simulink model "FAFA_Simulation"  (R2024b)
settings: Solver=FixedStepAuto  StartTime=0.0  StopTime=250  FixedStep=0.1  RelTol=1e-3
model workspace (MAT data in the model file):
  E = 0
  N = 0
  U = 70
  a_lat = [-2.8994 -3.7694 4.8979 0.9075 0.2017 1.1605 -2.4536 1.8506 -1.4522 0.9879 -4.2099 6.4665 ... (16 elements, 4x4)]
  a_lon = [-0.1636 0.8185 -0.1448 0.6823 -0.7164 -0.2899 -2.0395 -2.5415 0.3908 2.1971 -0.2446 -6.117 ... (16 elements, 4x4)]
  b_lat = [-2.6641  1.8404; -6.8743  1.3852; 17.3529  -0.0089; -11.8089  -3.3692]
  b_lon = [1.3105; 2.2437; -0.9608; -9.211]
  c_lat = [-0.6923 -1.1619 0.5476 -0.4273 0.0805 0.5751 0.4203 0.7792 -0.3221 1.1098 0.2079 0.2479 ... (16 elements, 4x4)]
  c_lon = [-5.1576 -0.0952 0.5331 3.6707 -28.9963 -0.3715 -3.4973 -0.1414 19.7487 -0.0997 -0.5832 -0.2256 ... (16 elements, 4x4)]
  d_lat = [0  0; 0  0; 0  0; 0  0]
  d_lon = [0; 0; 0; 0]
  psi0 = 0
  wind_E0 = 0
  wind_N0 = 0
  wind_heading = 100
  wind_noise = 0
  wind_turbulance_value0 = 1
  wind_value0 = 0
  x0_lat = [0; 0; 0; 0]
  x0_lon = [0; 0; 0; 0]
values from neighbouring files (symbols this model uses):
  velocity = zeros(num_waypoints, 3)    [training_engine.m]
  waypoints = all_waypoints    [training_engine.m]
undefined symbols (not defined in the file or in its folder): dspblkCoreblockFVToolHelper, F, gcbh, Light, MIL
libraries: simulink x8, slpidlib x5, aerolibwind2 x3, sharedtransform x2, rllib x1, uavutilslib x1
(part 2 of 3)

== matlab function FAFA_Simulation/OBSERVATION/MATLAB Function8 ==
  data: waypoints_window input; velocity_window input; valid_flag input; loiter_flag input; uav_e input; global_path output size=[inf 3]; uav_n input; uav_u input; guidance_mode output; uav_phi input; uav_theta input; uav_psi input
function [global_path, guidance_mode]   = guidance_function_hybrid(waypoints_window, velocity_window, valid_flag, loiter_flag, uav_e, uav_n, uav_u, uav_phi, uav_theta, uav_psi)

% guidance_mode: 0=無效, 1=純B-spline, 2=SPSO+B-spline, 3=Loiter模式

%#codegen

%  Loiter 模式開關
ENABLE_LOITER = false;

persistent last_point_initialized last_point stored_global_path stored_path_length ...
           loiter_mode initialized theta_current center loiter_arc transition

if isempty(last_point_initialized)
    last_point_initialized = false;
    last_point            = zeros(1,3);
    stored_global_path    = zeros(100000,3);
    stored_path_length    = 1;
    loiter_mode           = false;
    initialized = false;
    theta_current = 0;
    center = [0 0];
    loiter_arc = zeros(3,3);  % 固定初始大小
    transition = false;
end

% 確保 guidance_mode 在所有路徑都有明確的標量值
guidance_mode = 0;

R = 100;
dtheta_deg = 1;
uav_position = [uav_e, uav_n, uav_u];

%% ==== Loiter 模式 ====
% 只有當 ENABLE_LOITER = true 時才會進入 Loiter 邏輯
if ENABLE_LOITER && loiter_flag && ~initialized
    if stored_path_length >= 2
        pos_prev = stored_global_path(stored_path_length-1, 1:2);
        pos_curr = stored_global_path(stored_path_length, 1:2);
        heading_vec = pos_curr - pos_prev;
        yaw = atan2(heading_vec(2), heading_vec(1));
    else
        yaw = 0;
    end
    
    dists = vecnorm(waypoints_window(:,1:2) - uav_position(1:2), 2, 2);
    [~, idx_nearest] = min(dists);
    P0 = waypoints_window(idx_nearest, 1:2);
    center = P0 + [cos(yaw), sin(yaw)] * R * 1.5;
    theta_current = atan2(uav_position(2) - center(2), ...
                           uav_position(1) - center(1));
    loiter_mode = true;
    initialized = true;
end

if ENABLE_LOITER && loiter_mode
    guidance_mode = 3;
    if loiter_flag
        dtheta = deg2rad(dtheta_deg);
        spacing = 1.0;
        arc_length = R * dtheta;
        num_points = max(3, ceil(arc_length / spacing));
        theta_list = theta_current - linspace(0, dtheta, num_points);
        x_list = center(1) + R * cos(theta_list);
        y_list = center(2) + R * sin(theta_list);
        z_list = repmat(uav_u, size(x_list));

        loiter_arc_raw = [x_list', y_list', z_list'];
        arc_diff = diff(loiter_arc_raw);
        arc_seg_length = sqrt(sum(arc_diff.^2, 2));
        cum_length = [0; cumsum(arc_seg_length)];
        total_length = cum_length(end);

        num_interp = max(2, ceil(total_length));
        query_dist = linspace(0, total_length, num_interp)';
        interp_x = interp1(cum_length, loiter_arc_raw(:,1), query_dist, 'linear');
        interp_y = interp1(cum_length, loiter_arc_raw(:,2), query_dist, 'linear');
        interp_z = interp1(cum_length, loiter_arc_raw(:,3), query_dist, 'linear');
        loiter_arc = [interp_x, interp_y, interp_z];
        theta_current = theta_list(end);

        if ~transition
            loiter_entry = loiter_arc(1,:);
            loiter_tangent = loiter_arc(2,1:2) - loiter_arc(1,1:2);
            loiter_tangent = loiter_tangent / (norm(loiter_tangent) + 1e-6);

            dists = vecnorm(waypoints_window(:,1:2) - uav_position(1:2), 2, 2);
            [~, idx_nearest] = min(dists);
            P0 = waypoints_window(idx_nearest, :);
            
            connect_tangent = loiter_entry(1:2) - P0(1:2);
            connect_tangent = connect_tangent / (norm(connect_tangent) + 1e-6);
            dist = norm(loiter_entry(1:2) - P0(1:2));

            P1 = P0(1:2) + 0.3 * dist * connect_tangent;
            P2 = loiter_entry(1:2) - 0.3 * dist * loiter_tangent;
            P3 = loiter_entry(1:2);

            t = linspace(0,1,ceil(dist));
            bezier_x = (1-t).^3 * P0(1) + 3*(1-t).^2 .* t * P1(1) + 3*(1-t).*t.^2 * P2(1) + t.^3 * P3(1);
            bezier_y = (1-t).^3 * P0(2) + 3*(1-t).^2 .* t * P1(2) + 3*(1-t).*t.^2 * P2(2) + t.^3 * P3(2);
            bezier_z = linspace(P0(3), loiter_entry(3), numel(t));
            transition_path = [bezier_x', bezier_y', bezier_z'];

            combined_path = [transition_path; loiter_arc(2:end,:)];
            global_path = combined_path;
            transition = true;
        else
            global_path = loiter_arc;
        end
        return;
    else
        % 退出 Loiter 的邏輯
        arc_exit_pt = loiter_arc(end, :);
        arc_tangent = loiter_arc(end,1:2) - loiter_arc(end-1,1:2);
        arc_tangent = arc_tangent / (norm(arc_tangent) + 1e-6);
        R_min = 55;
        dists = vecnorm(waypoints_window(:,1:2) - arc_exit_pt(1:2), 2, 2);
        [~, idx_nearest] = min(dists);
        lookahead_distance = 100;
        accum_dist = 0;
        idx_target = idx_nearest;
        while accum_dist < lookahead_distance && idx_target < size(waypoints_window,1)
            delta = norm(waypoints_window(idx_target+1,1:2) - waypoints_window(idx_target,1:2));
            accum_dist = accum_dist + delta;
            idx_target = idx_target + 1;
        end
        p_target = waypoints_window(idx_target, :);
        if idx_target < size(waypoints_window,1)
            next_vec = waypoints_window(idx_target+1,1:2) - waypoints_window(idx_target,1:2);
        else
            next_vec = waypoints_window(idx_target,1:2) - waypoints_window(idx_target-1,1:2);
        end
        target_tangent = next_vec / (norm(next_vec) + 1e-6);
        P0 = arc_exit_pt;
        P3 = p_target;
        total_dist = norm(P3(1:2) - P0(1:2));
        theta = acos(dot(arc_tangent, target_tangent));
        d_min = R_min * tan(theta/2);
        d = max(d_min, R_min);
        success = false;
        B = repmat(P0, ceil(total_dist), 1);
        while ~success && d <= total_dist
            P1 = P0 + [arc_tangent, 0] * 0.3 * d;
            P2 = P3 - [target_tangent, 0] * 0.1 * d;
            t = linspace(0,1,ceil(total_dist));
            B = (1 - t').^3 * P0 + 3*(1 - t').^2 .* t' * P1 + 3*(1 - t') .* t'.^2 * P2 + t'.^3 * P3;
            d1 = diff(B, 1, 1);
            d2 = diff(d1, 1, 1);
            cross_z = d1(1:end-1,1) .* d2(:,2) - d1(1:end-1,2) .* d2(:,1);
            curvature = abs(cross_z) ./ (vecnorm(d1(1:end-1,:),2,2).^3 + 1e-6);
            if all(1./(curvature + 1e-6) >= R_min)
                success = true;
            else
                d = d + 5;
            end
        end
        segment = B;
        stored_global_path(1:size(segment,1), :) = segment;
        stored_path_length = size(segment,1);
        loiter_mode = false;
        initialized = false;
        transition = false;
        global_path = segment;
        % 固定維度賦值
        if size(segment,1) >= 1
            last_point(1,1) = segment(end, 1);
            last_point(1,2) = segment(end, 2);
            last_point(1,3) = segment(end, 3);
        end
        return;
    end
end

%% ========== v8 混合規劃器 ==========
if valid_flag && ~loiter_mode
    
    N_WAYPOINTS = size(waypoints_window, 1);
    
    % 起點處理 
    if ~last_point_initialized
        P_start_spline = [uav_e, uav_n, uav_u];
        last_point_initialized = true;
    else
        P_start_spline = last_point;
    end
    
    P_end = waypoints_window(end, :);

    % 判斷模式
    % dists_to_window = vecnorm(waypoints_window - uav_position, 2, 2);             % 三維距離
    dists_to_window = vecnorm(waypoints_window(:,1:2) - uav_position(1:2), 2, 2);   % 水平距離

    [min_dist_to_window, ~] = min(dists_to_window);
    % dist_start_to_window = norm(P_start_spline - waypoints_window(1,:));          % 三維距離
    dist_start_to_window = norm(P_start_spline(1:2) - waypoints_window(1,1:2));     % 水平距離

    DEVIATION_THRESHOLD = 100;  
    
    if min_dist_to_window < DEVIATION_THRESHOLD && dist_start_to_window < DEVIATION_THRESHOLD
        % ========== 模式A：純B-spline  ==========
        guidance_mode = 1;
        N_CONTROL_POINTS = 6;
        indices = round(linspace(1, N_WAYPOINTS, N_CONTROL_POINTS));
        best_control_points = waypoints_window(indices, :);
        best_control_points(1, :) = P_start_spline; 
    else
        % ========== 模式B：SPSO + B-spline ==========
        guidance_mode = 2;
        
        % SPSO 起點：強制為 UAV 當前位置
        P_start_SPSO = uav_position;
        
        % ====== 目標行駛方向（由速度滑窗估計，僅 SPSO 使用） ======
        v_tar_2d = [0, 0];
        if ~isempty(velocity_window)
            N_vel = size(velocity_window, 1);
            if N_vel >= 1
                K = min(3, N_vel);                    % 用最後 3 筆速度平均
                idx_start = N_vel - K + 1;
                v_seg = velocity_window(idx_start:N_vel, 1:2); % 只取 [vx, vy]
                v_mean = mean(v_seg, 1);
                if norm(v_mean) > 1e-3
                    v_tar_2d = v_mean;
                else
                    v_tar_2d = [0, 0];                % 速度太小則視為無效，不啟用角度限制
                end
            end
        end
        
        % SPSO參數
        nParticles = 10;
        maxIter = 20;
        w = 0.4;
        c1 = 1.5;
        c2 = 1.5;
        
        N_CONTROL_POINTS = 5; % 起點(UAV) + 3中間 + 終點
        N_OPTIMIZE = 3;
        
        % 定義 SPSO 粒子空間限制 (無人機運動學限制)
        % 直接限制粒子生成範圍
        max_segment_length = 50;
        min_segment_length = 5;
        max_climb_angle_rad = deg2rad(20); % 限制爬升角 theta
        % SPSO 粒子方位角相對轉角限制
        max_turn_angle_rad  = deg2rad(35); 
        
        % 權重設定 (總和 = 1)
        % b1: 路徑長度 (Shortest Path)
        % b2: 路徑跟隨 (Tracking)
        % b3: 平滑度 (Smoothness)
        % b4: 終點誤差 (Endpoint)
        b1 = 0.6; 
        b2 = 0.2; 
        b3 = 0.1; 
        b4 = 0.1; 

        % 參考採樣
        sample_idx = round(linspace(1, N_WAYPOINTS, N_CONTROL_POINTS));
        control_waypoints = waypoints_window(sample_idx, :);
        
        % 初始化參考向量 (基於 UAV 位置)
        reference_vectors = control_waypoints - P_start_SPSO;
        rho_ref = vecnorm(reference_vectors, 2, 2);
        theta_ref = asin(reference_vectors(:,3) ./ (rho_ref + 1e-6));
        phi_ref = atan2(reference_vectors(:,2), reference_vectors(:,1));
        
        dim = N_OPTIMIZE * 3;
        particles = zeros(nParticles, dim);
        velocities = zeros(nParticles, dim);
        
        for i = 1:nParticles
            for j = 1:N_OPTIMIZE
                ref_idx = j + 1;
                idx = (j-1)*3 + 1;
                
                if i == 1
                    % 第一個粒子用參考值
                    particles(1, idx)   = rho_ref(ref_idx);
                    particles(1, idx+1) = theta_ref(ref_idx);
                    particles(1, idx+2) = phi_ref(ref_idx);
                else
                    % 隨機生成
                    particles(i, idx)   = rho_ref(ref_idx) * (1 + randn() * 0.1);
                    particles(i, idx+1) = theta_ref(ref_idx) + randn() * deg2rad(2);
                    particles(i, idx+2) = phi_ref(ref_idx) + randn() * deg2rad(5);
                end
                
                % 在生成階段強制限制範圍
                % 限制長度 rho
                particles(i, idx) = max(min_segment_length, min(particles(i, idx), max_segment_length));
                % 限制爬升角 theta (直接對應無人機 Pitch/Climb 限制)
                particles(i, idx+1) = max(-max_climb_angle_rad, min(particles(i, idx+1), max_climb_angle_rad));
                
                % 限制方位角 phi 的「相對轉角」在 ±max_turn_angle_rad 內
                if j == 1
                    % 第一段以 UAV 目前航向為基準
                    base_heading = uav_psi;
                else
                    % 之後每一段以「前一段的 phi」為基準
                    prev_phi_idx = (j-2)*3 + 3;
                    base_heading = particles(i, prev_phi_idx);
                end
                dphi = particles(i, idx+2) - base_heading;
                % 將角度包回 [-pi, pi]
                dphi = mod(dphi + pi, 2*pi) - pi;
                % 夾住相對轉角
                if dphi > max_turn_angle_rad
                    dphi = max_turn_angle_rad;
                elseif dphi < -max_turn_angle_rad
                    dphi = -max_turn_angle_rad;
                end
                % 更新 phi 並保持在 [-pi, pi]
                particles(i, idx+2) = mod(base_heading + dphi + pi, 2*pi) - pi;
            end
            velocities(i, :) = randn(1, dim) * 0.01;
        end
        
        % SPSO迭代 - 初始 fitness
        fitness = zeros(nParticles, 1);
        for i = 1:nParticles
            % 傳入 uav_psi 以及 v_tar_2d 以計算初始航向與終端入射角
            fitness(i) = evaluateFitness_CostStruct(particles(i,:), P_start_SPSO, P_end, ...
                          control_waypoints, N_CONTROL_POINTS, b1, b2, b3, b4, ...
                          uav_psi, v_tar_2d);
        end
        
        [~, best_idx] = min(fitness);
        personal_best = particles;
        personal_best_fitness = fitness;
        global_best = particles(best_idx, :);
        global_best_fitness = fitness(best_idx);
        
        for iter = 1:maxIter
            for i = 1:nParticles
                r1 = rand(1, dim);
                r2 = rand(1, dim);
                velocities(i,:) = w * velocities(i,:) + ...
                                  c1 * r1 .* (personal_best(i,:) - particles(i,:)) + ...
                                  c2 * r2 .* (global_best - particles(i,:));
                particles(i,:) = particles(i,:) + velocities(i,:);
                
                % 更新後再次強制限制範圍 (Constraints)
                for j = 1:N_OPTIMIZE
                    idx = (j-1)*3 + 1;
                    % Rho Constraint
                    particles(i, idx) = max(min_segment_length, min(particles(i, idx), max_segment_length));
                    % Theta Constraint (Climb Angle)
                    particles(i, idx+1) = max(-max_climb_angle_rad, min(particles(i, idx+1), max_climb_angle_rad));
                    
                    % Phi Constraint: 限制每段方位角相對前一段 / UAV 航向的轉角
                    phi_idx = idx + 2;
                    if j == 1
                        base_heading = uav_psi;
                    else
                        prev_phi_idx = (j-2)*3 + 3;
                        base_heading = particles(i, prev_phi_idx);
                    end
                    dphi = particles(i, phi_idx) - base_heading;
                    % 將角度包回 [-pi, pi]
                    dphi = mod(dphi + pi, 2*pi) - pi;
                    % 夾住相對轉角
                    if dphi > max_turn_angle_rad
                        dphi = max_turn_angle_rad;
                    elseif dphi < -max_turn_angle_rad
                        dphi = -max_turn_angle_rad;
                    end
                    % 更新 phi 並保持在 [-pi, pi]
                    particles(i, phi_idx) = mod(base_heading + dphi + pi, 2*pi) - pi;
                end

                fitness(i) = evaluateFitness_CostStruct(particles(i,:), P_start_SPSO, P_end, ...
                              control_waypoints, N_CONTROL_POINTS, b1, b2, b3, b4, ...
                              uav_psi, v_tar_2d);

                if fitness(i) < personal_best_fitness(i)
                    personal_best(i,:) = particles(i,:);
                    personal_best_fitness(i) = fitness(i);
                end
            end
            
            [current_best_fitness, best_idx] = min(fitness);
            if current_best_fitness < global_best_fitness
                global_best = particles(best_idx, :);
                global_best_fitness = current_best_fitness;
            end
        end
        
        % 構建最終控制點
        best_control_points = zeros(N_CONTROL_POINTS, 3);
        best_control_points(1, :) = P_start_SPSO; 
        best_control_points(end, :) = P_end;
        for j = 1:N_OPTIMIZE
            idx = (j-1)*3 + 1;
            rho   = global_best(idx);
            theta = global_best(idx+1);
            phi   = global_best(idx+2);
            dx = rho * cos(theta) * cos(phi);
            dy = rho * cos(theta) * sin(phi);
            dz = rho * sin(theta);
            best_control_points(j+1, :) = best_control_points(j, :) + [dx, dy, dz];
        end
    end
    
    % 生成 B-spline
    N_samples = 100;
    path_smooth = generate_Bspline(best_control_points, N_samples);
    
    % Resample
    segment_diff = diff(path_smooth);
    segment_length = sqrt(sum(segment_diff.^2, 2));
    cumulative_length = [0; cumsum(segment_length)];
    total_length = cumulative_length(end);
    
    if total_length < 1e-3
        if stored_path_length > 1
             global_path = stored_global_path(1:stored_path_length,:);
        else
             global_path = path_smooth;
        end
        return;
    end
    
    desired_spacing = 1;
    num_new_points = max(2, floor(total_length / desired_spacing));
    query_distances = linspace(0, total_length, num_new_points)';
    
    interp_x = interp1(cumulative_length, path_smooth(:,1), query_distances, 'linear');
    interp_y = interp1(cumulative_length, path_smooth(:,2), query_distances, 'linear');
    interp_z = interp1(cumulative_length, path_smooth(:,3), query_distances, 'linear');
    
    new_path = [interp_x, interp_y, interp_z];
    stored_global_path(:,:) = 0;
    if isempty(new_path)
        stored_global_path(1:size(best_control_points,1),:) = best_control_points;
        stored_path_length = size(best_control_points,1);
        % 固定維度賦值
        last_point(1,1) = best_control_points(end, 1);
        last_point(1,2) = best_control_points(end, 2);
        last_point(1,3) = best_control_points(end, 3);
    else
        stored_global_path(1:size(new_path,1),:) = new_path;
        stored_path_length = size(new_path,1);
        % 固定維度賦值
        last_point(1,1) = new_path(end, 1);
        last_point(1,2) = new_path(end, 2);
        last_point(1,3) = new_path(end, 3);
    end
end

global_path = stored_global_path(1:stored_path_length,:);
end

%% ========== B-spline生成器 ==========
function path_smooth = generate_Bspline(control_points, num_samples)
    N = size(control_points, 1);
    if N < 2
        path_smooth = control_points;
        return;
    end
    segment_lengths = sqrt(sum(diff(control_points).^2, 2));
    t_control = [0; cumsum(segment_lengths)];
    valid_idx = [true; segment_lengths > 1e-6];
    if sum(valid_idx) < 2
        path_smooth = repmat(control_points(1,:), num_samples, 1);
        return;
    end
    t_control_valid = t_control(valid_idx);
    control_points_valid = control_points(valid_idx, :);
    if isempty(t_control_valid) || t_control_valid(end) < 1e-6
        path_smooth = repmat(control_points(1,:), num_samples, 1);
        return;
    end
    t_control_valid = t_control_valid / t_control_valid(end); 
    t_query = linspace(0, 1, num_samples)';
    x_smooth = spline(t_control_valid, control_points_valid(:,1), t_query);
    y_smooth = spline(t_control_valid, control_points_valid(:,2), t_query);
    z_smooth = spline(t_control_valid, control_points_valid(:,3), t_query);
    path_smooth = [x_smooth, y_smooth, z_smooth];
end

%% ========== Cost Function（含終端入射角約束） ==========
function cost = evaluateFitness_CostStruct(particle, P_start, P_end, control_waypoints, N_control, ...
                                           b1, b2, b3, b4, ...
                                           uav_psi, v_tar_2d)
    % particle: SPSO 粒子向量
    % b1: Shortest Path (長度)
    % b2: Tracking (跟隨誤差)
    % b3: Smoothness (平滑度 & 初始姿態限制)
    % b4: Endpoint (終點誤差)
    % v_tar_2d: 目標行駛方向（由速度滑窗估計）[vx, vy]
    
    % 1. 重建路徑 (SPSO 控制點)
    path = zeros(N_control, 3);
    path(1, :) = P_start;
    path(end, :) = P_end;
    
    N_optimize = (N_control - 2);
    for j = 1:N_optimize
        idx = (j-1)*3 + 1;
        rho   = particle(idx);
        theta = particle(idx+1);
        phi   = particle(idx+2);
        dx = rho * cos(theta) * cos(phi);
        dy = rho * cos(theta) * sin(phi);
        dz = rho * sin(theta);
        path(j+1, :) = path(j, :) + [dx, dy, dz];
    end
    
    % ========== F1: 路徑長度成本 (Shortest Path) ==========
    path_diff = diff(path);
    segment_lengths = sqrt(sum(path_diff.^2, 2));
    total_length = sum(segment_lengths);
    straight_dist = norm(P_end - P_start);
    
    if straight_dist > 1e-6
        F1 = total_length / straight_dist; % 越接近1越好
        F1 = min(F1, 3.0); % 上限截斷
    else
        F1 = 1.0;
    end
    
    % ========== F2: 路徑跟隨成本 (Tracking) ==========
    F2_raw = 0;
    for i = 1:size(path,1)
        dists = vecnorm(control_waypoints - path(i,:), 2, 2);
        [min_dist, ~] = min(dists);
        F2_raw = F2_raw + min_dist^2; % 平方懲罰
    end
    F2 = F2_raw / (size(path,1) * 100); % 簡單歸一化
    F2 = min(F2, 10.0);

    % ========== F3: 平滑度成本 (Smoothness & UAV Heading) ==========
    F3_raw = 0;
    max_turn_angle = deg2rad(35);
    
    % (A) 檢查第一段路徑與 UAV 當前航向 (psi) 的夾角
    vec_first = path(2,1:2) - path(1,1:2);
    if norm(vec_first) > 1e-6
        current_psi_vec = [cos(uav_psi), sin(uav_psi)];
        dot_val = dot(vec_first/norm(vec_first), current_psi_vec);
        angle_diff_start = acos(max(-1, min(1, dot_val)));
        
        % 如果起步轉彎大於限制，給予巨大懲罰
        if angle_diff_start > max_turn_angle
            cost = 1e9; 
            return;
        end
        F3_raw = F3_raw + angle_diff_start;
    end
    
    % (B) 檢查後續路徑段之間的夾角
    for i = 1:size(path,1)-2
        v1 = path(i+1,1:2) - path(i,1:2);
        v2 = path(i+2,1:2) - path(i+1,1:2);
        
        if norm(v1) > 1e-6 && norm(v2) > 1e-6
            dot_prod = dot(v1, v2);
            cross_prod = v1(1)*v2(2) - v1(2)*v2(1);
            phi_turn = atan2(cross_prod, dot_prod);
            
            if abs(phi_turn) > max_turn_angle
                cost = 1e9;
                return;
            end
            F3_raw = F3_raw + abs(phi_turn);
        end
    end
    F3 = F3_raw; % 可根據需要添加歸一化因子
    
    % ========== F4: 終點誤差成本 (Endpoint) ==========
    endpoint_error = norm(path(end,:) - P_end);
    if endpoint_error > 20 % 硬約束寬鬆一點給 SPSO
        cost = 1e9 + endpoint_error * 1000;
        return;
    end
    F4 = endpoint_error / 10.0;
    
    % ========== F5: 終端入射角成本（硬約束：±45°） ==========
    % 僅當 v_tar_2d 有效時啟用（速度非接近 0）
    if ~(v_tar_2d(1) == 0 && v_tar_2d(2) == 0)
        if size(path,1) < 2
            cost = 1e9;
            return;
        end
        
        % 終端路徑的切線向量（水平平面）
        v_last = path(end,1:2) - path(end-1,1:2);
        if norm(v_last) < 1e-6
            cost = 1e9;
            return;
        end
        v_last = v_last / norm(v_last);
        
        % 目標行駛方向向量正規化
        v_tar = v_tar_2d;
        if norm(v_tar) < 1e-6
            % 如果這裡還是太小，就不啟用此約束
        else
            v_tar = v_tar / norm(v_tar);
            
            % 入射角：終端切線 vs 目標行駛方向
            dot_val   = dot(v_last, v_tar);
            dot_val   = max(-1, min(1, dot_val));
            cross_val = v_last(1)*v_tar(2) - v_last(2)*v_tar(1);
            delta_psi_entry = atan2(cross_val, dot_val);  % [-pi, pi]
            
            max_entry = deg2rad(45); % 入射角限制 ±45°
            if abs(delta_psi_entry) > max_entry
                cost = 1e9;
                return;
            end
        end
    end

    % ========== 總成本 ==========
    cost = b1*F1 + b2*F2 + b3*F3 + b4*F4;
    
    if isnan(cost) || isinf(cost)
        cost = 1e10;
    end
end

== matlab function FAFA_Simulation/OBSERVATION/MATLAB Function10 ==
  data: x input; y output; finite input
function y = Normalization(x,finite)
y = (x-(-finite))/(finite-(-finite))*2-1;

== matlab function FAFA_Simulation/OBSERVATION/MATLAB Function9 ==
  data: x input; y output; finite input
function y = Normalization(x,finite)
y = (x-(-finite))/(finite-(-finite))*2-1;

== matlab function FAFA_Simulation/OBSERVATION/MATLAB Function13 ==
  data: kt input; y output; d input
function y = fcn(kt, d)

if abs(kt) >= (1/55)
    y = 0.5 *d;
else
    y = d;
end

== matlab function FAFA_Simulation/OBSERVATION/MATLAB Function11 ==
  data: x input; y output; finite input
function y = Normalization(x,finite)
y = (x-(-finite))/(finite-(-finite))*2-1;

== matlab function FAFA_Simulation/OBSERVATION/MATLAB Function12 ==
  data: E output; P_N input; N output; P_E input; psi input; v input; path input; d output; delta_psi output; heta output; curvature output; windowLen input
function [E, N, d, delta_psi, heta, curvature] = guidance_law(P_N, P_E, psi, v, path, windowLen)

    persistent global_path path_length last_path old_length heta_filt
    
    if isempty(global_path)
        global_path = zeros(500000, 3);
        path_length = 0;
        last_path = zeros(500000, 3);
        old_length = 0;
        heta_filt = 0;
    end
    
    % 如果這次輸入的 path 不等於上次的，就加入累積
    if ~isempty(path) && ~isequal(path, last_path(1:old_length, :))
        new_len = size(path, 1);
        global_path(path_length+1:path_length+new_len, :) = path(:, :);
        path_length = path_length + new_len;
        last_path(1:new_len, :) = path(:, :);
        old_length = new_len;
    end
    path_CTE = global_path(1:path_length, :);

    r = 0;
    curvature = 0;
    d = 0;
    delta_psi = 0;
    heta = 0;

    % Use the waypoints in the given path
    numWps = size(path, 1);
    if numWps < 2
        N = P_N;
        E = P_E;
        return;
    end

    % ============================================================
    % 前瞻曲率（用滑窗 path 末端那一段來估）
    % ============================================================
    if numWps < 3
        curvature = 0;
    else
        % 調這兩個 
        previewDist = 0.9 * windowLen;  % 看視野最前端附近（90%處） 300*0.9=270
        spanDist    = max(10, 0.1 * windowLen); % 用 10%視野估曲率，至少10m,270*0.1=27,計算270m前後27m的曲率
        % ------------------------

        % 以 path 起點為 0，計算沿路徑累積距離（平面 E,N）
        xy = path(:,1:2);
        s  = [0; cumsum(sqrt(sum(diff(xy).^2,2)))];  % s(i) = 第 i 點距離 path(1) 的弧長
        L  = s(end);

        if L < 1e-6
            curvature = 0;
        else
            % 把 previewDist 限制在滑窗長度內
            s2 = min(max(previewDist, 0), L);
            s1 = max(s2 - spanDist/2, 0);
            s3 = min(s2 + spanDist/2, L);

            % 找到最接近 s1,s2,s3 的三個點索引
            [~, i1] = min(abs(s - s1));
            [~, i2] = min(abs(s - s2));
            [~, i3] = min(abs(s - s3));

            % 確保三點不重疊（避免除0）
            if numel(unique([i1 i2 i3])) < 3
                curvature = 0;
            else
                A = xy(i1,:); B = xy(i2,:); C = xy(i3,:);

                a = norm(B - C);
                b = norm(A - C);
                c = norm(A - B);

                % signed area2 = 2*Area (帶正負號可分左右轉)
                area2 = (B(1)-A(1))*(C(2)-A(2)) - (B(2)-A(2))*(C(1)-A(1));

                if a*b*c < 1e-9 || abs(area2) < 1e-9
                    curvature = 0;
                    r = 0;
                else
                    curvature = (2 * area2) / (a*b*c);   % signed curvature (1/m)
                    r = 1 / max(abs(curvature), 1e-9);
                end
            end
        end
    end
    % ============================================================

    margin = 30;  
    min_E = min(path(:,1)) - margin;
    max_E = max(path(:,1)) + margin;
    min_N = min(path(:,2)) - margin;
    max_N = max(path(:,2)) + margin;

    is_inside = (P_E >= min_E) && (P_E <= max_E) && ...
            (P_N >= min_N) && (P_N <= max_N);

    if is_inside
        extended_P = repmat([P_E, P_N], numWps, 1);
        differences = path(:, 1:2) - extended_P;
        distances = sqrt(sum(differences.^2, 2));
        
        % Find the closest waypoint
        [~, current_index] = min(distances);
        
        % Define target distance
        target_distance = 50;
        
        % Compute cumulative distances
        cumulative_distances = [0; cumsum(sqrt(sum(diff(path).^2, 2)))];
        remaining_distances = cumulative_distances(current_index+1:end) - cumulative_distances(current_index);
        
        % Determine target index
        if isempty(remaining_distances) || current_index + 1 > numWps
            k = numWps;
        else
            % Find the waypoint at the target distance
            [~, target_index_offset] = min(abs(remaining_distances - target_distance));
            
            if current_index + target_index_offset > numWps
                k = numWps;
            else
                k = current_index + target_index_offset;
            end
        end
        
        % Target waypoint
        N = path(k, 2); 
        E = path(k, 1); 
    
        % Compute cross-track error
        if current_index >= numWps
            x1 = path(numWps-1, 1);
            y1 = path(numWps-1, 2);
            x2 = path(numWps, 1);
            y2 = path(numWps, 2);
        else
            x1 = path(current_index, 1);
            y1 = path(current_index, 2);
            x2 = path(current_index+1, 1);
            y2 = path(current_index+1, 2);
        end
        
        D = sqrt((P_N - y1)^2 + (P_E - x1)^2);
        psi_r = atan2(y2 - y1, x2 - x1);
        psi_c = atan2(P_N - y1, P_E - x1);
    
        if abs(psi_r - psi_c) < 1e-3
            d = 0; % 避免極小角度導致大誤差
        else
            d = abs(D * sin(psi_r - psi_c));
        end
           
        % Evaluation candidate: extend terminal lookahead while waiting for a new path.
        % Only the inside-window branch and its endpoint target are affected.
        if k == numWps
            tail = path(numWps,1:2) - path(numWps-1,1:2);
            tail_length = norm(tail);
            if tail_length > 1e-6
                tangent = tail / tail_length;
                along = dot([P_E, P_N] - path(numWps,1:2), tangent);
                extension = max(0, target_distance + along);
                E = path(numWps,1) + extension*tangent(1);
                N = path(numWps,2) + extension*tangent(2);
            end
        end

        % Compute heading difference
        psi_cmd = atan2(N - P_N, E - P_E);
        heta = psi_cmd - psi;
        heta = mod(heta + pi, 2 * pi) - pi;
    
        L1 = sqrt((N - P_N)^2 + (E - P_E)^2);
        a_cmd = 2 * v^2 / L1 * sin(heta);
        delta_psi = a_cmd / v;

    else  % ~is_inside
        
        numWaypoints = size(path_CTE, 1);
        % Calculate distances to all waypoints
        extended_P = repmat([P_E, P_N], numWaypoints, 1);
        differences = path_CTE(:, 1:2) - extended_P;
        distances = sqrt(sum(differences.^2, 2));
        
        % Find the closest waypoint
        [~, current_index] = min(distances);
        
        % Define target distance
        target_distance = 30;
        uav_pos = [P_E, P_N];
        path_points = path(:,1:2);
        point_dists = vecnorm(path_points - uav_pos, 2, 2);
        [~, k] = min(abs(point_dists - target_distance));
        
        % Target waypoint
        E = path(k, 1); 
        N = path(k, 2); 
    
        % Compute cross-track error
        if current_index >= numWaypoints
            x1 = path_CTE(numWaypoints-1, 1);
            y1 = path_CTE(numWaypoints-1, 2);
            x2 = path_CTE(numWaypoints, 1);
            y2 = path_CTE(numWaypoints, 2);
        else
            x1 = path_CTE(current_index, 1);
            y1 = path_CTE(current_index, 2);
            x2 = path_CTE(current_index+1, 1);
            y2 = path_CTE(current_index+1, 2);
        end
        
        D = sqrt((P_N - y1)^2 + (P_E - x1)^2);
        psi_r = atan2(y2 - y1, x2 - x1);
        psi_c = atan2(P_N - y1, P_E - x1);
    
        if abs(psi_r - psi_c) < 1e-3
            d = 0; % 避免極小角度導致大誤差
        else
            d = abs(D * sin(psi_r - psi_c));
        end
    
        % V2: only handle longitudinal overshoot near the terminal ray.
        tail = path(numWps,1:2) - path(numWps-1,1:2);
        tail_length = norm(tail);
        if tail_length > 1e-6
            tangent = tail / tail_length;
            offset = [P_E, P_N] - path(numWps,1:2);
            along = dot(offset, tangent);
            lateral = norm(offset - along*tangent);
            [~, nearest_terminal] = min(point_dists);
            if nearest_terminal == numWps && along >= 0 && lateral <= margin
                E = path(numWps,1) + (along + 50)*tangent(1);
                N = path(numWps,2) + (along + 50)*tangent(2);
            end
        end

        % Compute heading difference
        psi_cmd = atan2(N - P_N, E - P_E);
        heta = psi_cmd - psi;
        heta = mod(heta + pi, 2 * pi) - pi;
        if heta_filt == 0
            heta_filt = heta;
        end
        alpha = 0.85;
       
        heta_filt = alpha * heta_filt + (1 - alpha) * heta;
        heta = heta_filt;
    
        L1 = sqrt((N - P_N)^2 + (E - P_E)^2);
        a_cmd = 2 * v^2 / L1 * sin(heta);
        delta_psi = a_cmd / v;
    end
end

== matlab function FAFA_Simulation/OBSERVATION/MATLAB Function15 ==
  data: x input; y output; finite input
function y = Normalization(x,finite)
y = (x-(-finite))/(finite-(-finite))*2-1;

== matlab function FAFA_Simulation/OBSERVATION/MATLAB Function14 ==
  data: d input; dis input; y output
function y = fcn(d, dis)
    if isempty(dis)
        y = 0;
    end
    if dis <= 150 && dis >= 30
        a = 0.5;
    else
        a = 0;
    end
    if d <= 10
        b = 0.5;
    else
        b = 0;
    end
    y = a+b;

end

== matlab function FAFA_Simulation/OBSERVATION/MATLAB Function16 ==
  data: roll input; r_roll output; roll_d input
function r_roll  = fcn(roll,roll_d)
roll_dot = (roll-roll_d)/0.1;

% ele_dot = (ele-ele_d)/0.1;
if abs(roll_dot)>6
    r_roll = -0.1;
else
    r_roll = 0;
end

% if abs(ele_dot)>6
%     r_ele = -0.1;
% else
%     r_ele = 0;
% end

== matlab function FAFA_Simulation/OBSERVATION/MATLAB Function18 ==
  data: x input; y output; Finite input
function y = Normalization(x,Finite)

y = (x-(-Finite))/(Finite-(-Finite))*2-1;
